simulink model "Factory_Physics_Model"  (R2024b)
settings: Solver=ode4  StartTime=0  StopTime=120  FixedStep=0.0005  RelTol=1e-3
model workspace (MAT data in the model file):
  FACTORY_EXT_CMD = 0
settings Model: Creator=shash  LastModifiedBy=shash
settings ModelReferenceCC: ModelReferenceNumInstancesAllowed=Single

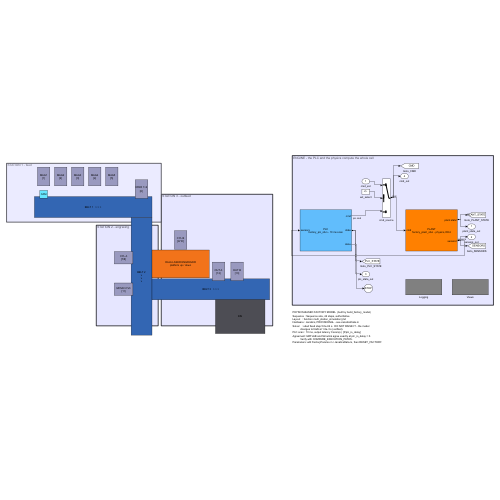
[thumbnail: Simulink's stored preview of the top-level diagram]
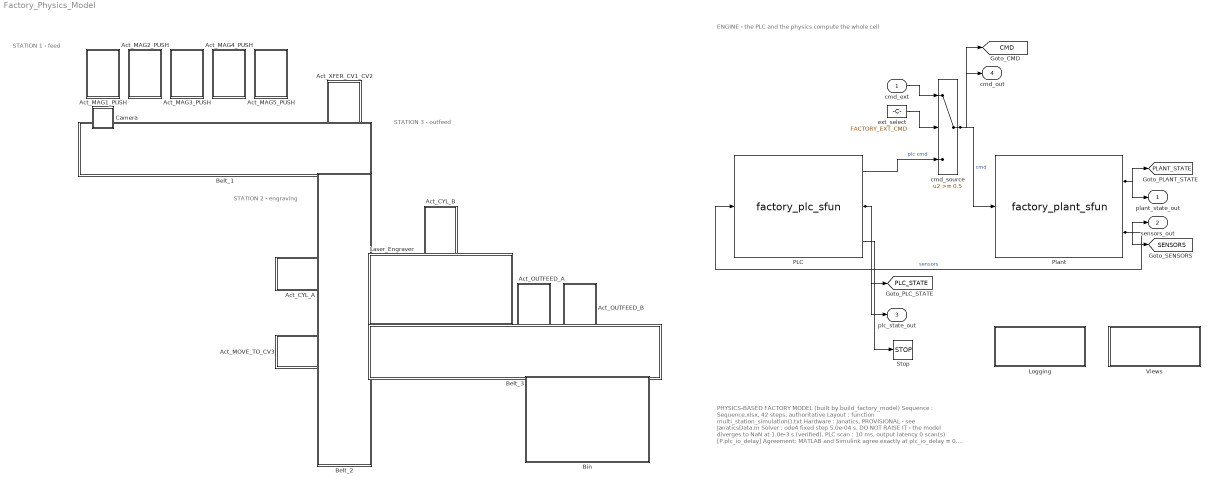
== system Factory_Physics_Model ==
  note: PHYSICS-BASED FACTORY MODEL  (built by build_factory_model)
      | Sequence : Sequence.xlsx, 42 steps, authoritative
      | Layout   : function multi_station_simulation().txt
      | Hardware : Janatics, PROVISIONAL - see JanaticsData.m
      | Solver   : ode4 fixed step 5.0e-04 s.  DO NOT RAISE IT - the model
      |            diverges to NaN at 1.0e-3 s (verified).
      | PLC scan : 10 ms, output latency 0 scan(s)  [P.plc_io_delay]
      | Agreement: MATLAB and Simulink agree exactly at plc_io_delay = 0.
      |            Verify with COMPARE_EXECUTION_PATHS.
      | Parameters: edit FactoryParams.m / JanaticsData.m, then RESET_FACTORY.
  note: STATION 1 - feed
  note: STATION 2 - engraving
  note: STATION 3 - outfeed
  note: ENGINE - the PLC and the physics compute the whole cell
  cmd_ext : Inport  PortDimensions=22
  Act_CYL_A : Subsystem
      mask Display: disp('CYL A\n[7/8]');
  Act_CYL_B : Subsystem
      mask Display: disp('CYL B\n[9/10]');
  Act_MAG1_PUSH : Subsystem
      mask Display: disp('MAG1\n[1]');
  Act_MAG2_PUSH : Subsystem
      mask Display: disp('MAG2\n[2]');
  Act_MAG3_PUSH : Subsystem
      mask Display: disp('MAG3\n[3]');
  Act_MAG4_PUSH : Subsystem
      mask Display: disp('MAG4\n[4]');
  Act_MAG5_PUSH : Subsystem
      mask Display: disp('MAG5\n[5]');
  Act_MOVE_TO_CV3 : Subsystem
      mask Display: disp('MOVE>CV3\n[11]');
  Act_OUTFEED_A : Subsystem
      mask Display: disp('OUT A\n[12]');
  Act_OUTFEED_B : Subsystem
      mask Display: disp('OUT B\n[13]');
  Act_XFER_CV1_CV2 : Subsystem
      mask Display: disp('XFER 1>2\n[6]');
  Belt_1 : Subsystem
      mask Display: disp('BELT 1   > > >');
  Belt_2 : Subsystem
      mask Display: disp('BELT 2\nv\nv\nv');
  Belt_3 : Subsystem
      mask Display: disp('BELT 3   > > >');
  Bin : Subsystem
      mask Display: disp('BIN');
  Camera : Subsystem
      mask Display: disp('CAM');
  Laser_Engraver : Subsystem
      mask Display: disp('DAJA LASER ENGRAVER\nplatform up / down');
  Logging : Subsystem
  PLC : M-S-Function  FunctionName=factory_plc_sfun
      mask Display:
      | disp('PLC\nfactory_plc_sfun - 10 ms scan');
      | port_label('input', 1, 'sensors');
      | port_label('output', 1, 'cmd');
      | port_label('output', 2, 'state');
      | port_label('output', 3, 'done');
  Plant : M-S-Function  FunctionName=factory_plant_sfun
      mask Display:
      | disp('PLANT\nfactory_plant_sfun - physics, RK4');
      | port_label('input', 1, 'cmd');
      | port_label('output', 1, 'plant state');
      | port_label('output', 2, 'sensors');
  Stop : Stop
  Views : Subsystem
  cmd_source : Switch  Threshold=0.5
  ext_select : Constant  Value=FACTORY_EXT_CMD
  plant_state_out : Outport
  sensors_out : Outport  Port=2
  plc_state_out : Outport  Port=3
  cmd_out : Outport  Port=4
  tag scope: CMD=global, PLANT_STATE=global, PLC_STATE=global, SENSORS=global
  wires:
  cmd_ext/1 -> cmd_source/1
  ext_select/1 -> cmd_source/2
  PLC/1 -> cmd_source/3  "plc cmd"
  cmd_source/1 -> Plant/1, [CMD], cmd_out/1  "cmd"
  Plant/2 -> PLC/1, [SENSORS], sensors_out/1  "sensors"
  PLC/3 -> Stop/1
  Plant/1 -> [PLANT_STATE], plant_state_out/1
  PLC/2 -> [PLC_STATE], plc_state_out/1

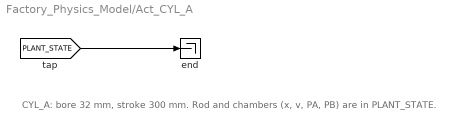
== system Factory_Physics_Model/Act_CYL_A ==
  note: CYL_A: bore 32 mm, stroke 300 mm. Rod and chambers (x, v, PA, PB) are in PLANT_STATE.
  end : Terminator
  wires:
  [PLANT_STATE] -> end/1

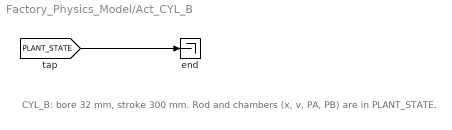
== system Factory_Physics_Model/Act_CYL_B ==
  note: CYL_B: bore 32 mm, stroke 300 mm. Rod and chambers (x, v, PA, PB) are in PLANT_STATE.
  end : Terminator
  wires:
  [PLANT_STATE] -> end/1

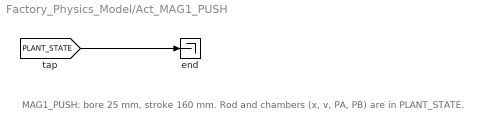
== system Factory_Physics_Model/Act_MAG1_PUSH ==
  note: MAG1_PUSH: bore 25 mm, stroke 160 mm. Rod and chambers (x, v, PA, PB) are in PLANT_STATE.
  end : Terminator
  wires:
  [PLANT_STATE] -> end/1

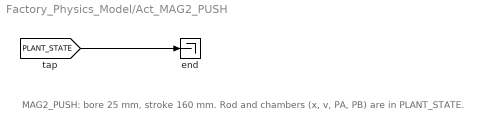
== system Factory_Physics_Model/Act_MAG2_PUSH ==
  note: MAG2_PUSH: bore 25 mm, stroke 160 mm. Rod and chambers (x, v, PA, PB) are in PLANT_STATE.
  end : Terminator
  wires:
  [PLANT_STATE] -> end/1

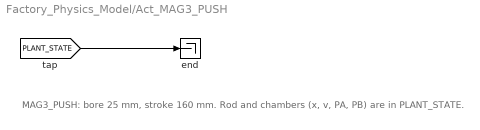
== system Factory_Physics_Model/Act_MAG3_PUSH ==
  note: MAG3_PUSH: bore 25 mm, stroke 160 mm. Rod and chambers (x, v, PA, PB) are in PLANT_STATE.
  end : Terminator
  wires:
  [PLANT_STATE] -> end/1

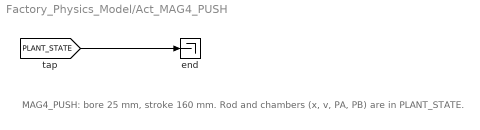
== system Factory_Physics_Model/Act_MAG4_PUSH ==
  note: MAG4_PUSH: bore 25 mm, stroke 160 mm. Rod and chambers (x, v, PA, PB) are in PLANT_STATE.
  end : Terminator
  wires:
  [PLANT_STATE] -> end/1

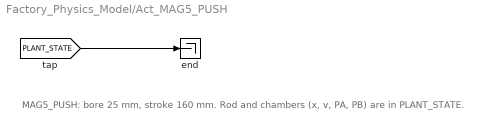
== system Factory_Physics_Model/Act_MAG5_PUSH ==
  note: MAG5_PUSH: bore 25 mm, stroke 160 mm. Rod and chambers (x, v, PA, PB) are in PLANT_STATE.
  end : Terminator
  wires:
  [PLANT_STATE] -> end/1

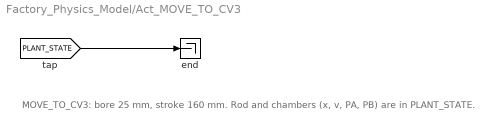
== system Factory_Physics_Model/Act_MOVE_TO_CV3 ==
  note: MOVE_TO_CV3: bore 25 mm, stroke 160 mm. Rod and chambers (x, v, PA, PB) are in PLANT_STATE.
  end : Terminator
  wires:
  [PLANT_STATE] -> end/1

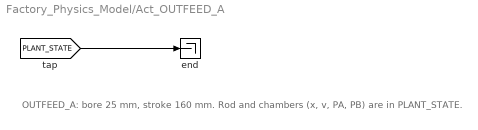
== system Factory_Physics_Model/Act_OUTFEED_A ==
  note: OUTFEED_A: bore 25 mm, stroke 160 mm. Rod and chambers (x, v, PA, PB) are in PLANT_STATE.
  end : Terminator
  wires:
  [PLANT_STATE] -> end/1

== system Factory_Physics_Model/Act_OUTFEED_B ==
  note: OUTFEED_B: bore 25 mm, stroke 160 mm. Rod and chambers (x, v, PA, PB) are in PLANT_STATE.
  end : Terminator
  wires:
  [PLANT_STATE] -> end/1

== system Factory_Physics_Model/Act_XFER_CV1_CV2 ==
  note: XFER_CV1_CV2: bore 25 mm, stroke 160 mm. Rod and chambers (x, v, PA, PB) are in PLANT_STATE.
  end : Terminator
  wires:
  [PLANT_STATE] -> end/1

== system Factory_Physics_Model/Belt_1 ==
  note: Conveyor 1. Its drive states (om, ei, vref) are in PLANT_STATE; open Views for scopes.
  end : Terminator
  wires:
  [PLANT_STATE] -> end/1

== system Factory_Physics_Model/Belt_2 ==
  note: Conveyor 2, into the engraver. Drive states in PLANT_STATE.
  end : Terminator
  wires:
  [PLANT_STATE] -> end/1

== system Factory_Physics_Model/Belt_3 ==
  note: Conveyor 3, to the outfeed. Drive states in PLANT_STATE.
  end : Terminator
  wires:
  [PLANT_STATE] -> end/1

== system Factory_Physics_Model/Bin ==
  note: Collection bin, fed by both outfeed pushers.
  end : Terminator
  wires:
  [SENSORS] -> end/1

== system Factory_Physics_Model/Camera ==
  note: The camera that detects the part (CAM, sensor index 1).
  end : Terminator
  wires:
  [SENSORS] -> end/1

== system Factory_Physics_Model/Laser_Engraver ==
  note: Platform up (S23), laser and ENG DONE (S24-S26), platform down (S27-S28).
  end : Terminator
  wires:
  [PLC_STATE] -> end/1

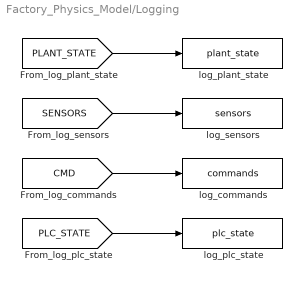
== system Factory_Physics_Model/Logging ==
  log_commands : ToWorkspace  VariableName=commands  SaveFormat=Structure With Time
      settings: Decimation=20
  log_plant_state : ToWorkspace  VariableName=plant_state  SaveFormat=Structure With Time
      settings: Decimation=20
  log_plc_state : ToWorkspace  VariableName=plc_state  SaveFormat=Structure With Time
      settings: Decimation=20
  log_sensors : ToWorkspace  VariableName=sensors  SaveFormat=Structure With Time
      settings: Decimation=20
  wires:
  [PLANT_STATE] -> log_plant_state/1
  [SENSORS] -> log_sensors/1
  [CMD] -> log_commands/1
  [PLC_STATE] -> log_plc_state/1

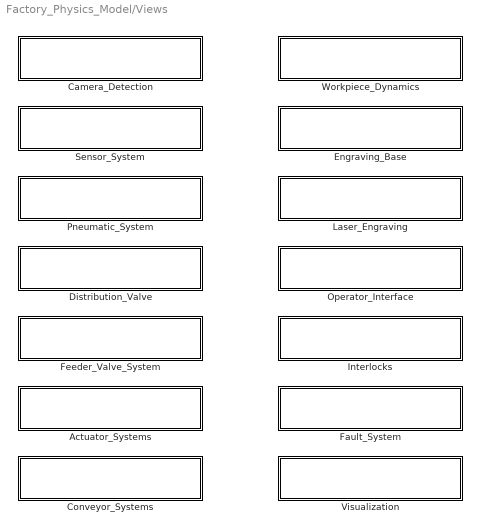
== system Factory_Physics_Model/Views ==
  Actuator_Systems : Subsystem
  Camera_Detection : Subsystem
  Conveyor_Systems : Subsystem
  Distribution_Valve : Subsystem
  Engraving_Base : Subsystem
  Fault_System : Subsystem
  Feeder_Valve_System : Subsystem
  Interlocks : Subsystem
  Laser_Engraving : Subsystem
  Operator_Interface : Subsystem
  Pneumatic_System : Subsystem
  Sensor_System : Subsystem
  Visualization : Subsystem
  Workpiece_Dynamics : Subsystem

== system Factory_Physics_Model/Views/Actuator_Systems ==
  note: PA 10:20, PB 21:31, x 32:42, v 43:53
  view : Scope
  wires:
  [PLANT_STATE] -> view/1

== system Factory_Physics_Model/Views/Camera_Detection ==
  note: CAM = index 1
  view : Scope
  wires:
  [SENSORS] -> view/1

== system Factory_Physics_Model/Views/Conveyor_Systems ==
  note: om 65:67, ei 68:70, vref 71:73
  view : Scope
  wires:
  [PLANT_STATE] -> view/1

== system Factory_Physics_Model/Views/Distribution_Valve ==
  note: dv 6:9
  view : Scope
  wires:
  [PLANT_STATE] -> view/1

== system Factory_Physics_Model/Views/Engraving_Base ==
  note: bz 74, bvz 75, bei 76
  view : Scope
  wires:
  [PLANT_STATE] -> view/1

== system Factory_Physics_Model/Views/Fault_System ==
  note: switches live in P.fault, not in the diagram
  view : Scope
  wires:
  [PLANT_STATE] -> view/1

== system Factory_Physics_Model/Views/Feeder_Valve_System ==
  note: sp 54:64
  view : Scope
  wires:
  [PLANT_STATE] -> view/1

== system Factory_Physics_Model/Views/Interlocks ==
  note: P_READY 37, BR_RDY 38:41, CHG 42:52
  view : Scope
  wires:
  [SENSORS] -> view/1

== system Factory_Physics_Model/Views/Laser_Engraving ==
  note: states 25..29 are the engraving process
  view : Scope
  wires:
  [PLC_STATE] -> view/1

== system Factory_Physics_Model/Views/Operator_Interface ==
  note: states 25,26,27 - PLACEHOLDER timings
  view : Scope
  wires:
  [PLC_STATE] -> view/1

== system Factory_Physics_Model/Views/Pneumatic_System ==
  note: P_res 1, P_br 2:5
  view : Scope
  wires:
  [PLANT_STATE] -> view/1

== system Factory_Physics_Model/Views/Sensor_System ==
  note: PX 2:11, EXT 12:22, RET 23:33, HS_TOP 34, HS_BOT 35
  view : Scope
  wires:
  [SENSORS] -> view/1

== system Factory_Physics_Model/Views/Visualization ==
  note: use visualize_factory(LOG) from MATLAB
  view : Scope
  wires:
  [PLANT_STATE] -> view/1

== system Factory_Physics_Model/Views/Workpiece_Dynamics ==
  note: bx 77, by 78, bvx 79, bvy 80
  view : Scope
  wires:
  [PLANT_STATE] -> view/1
